simulink model "robot_2int_PI"  (R2024b)
settings: Solver=VariableStepAuto  StartTime=0.0  StopTime=10  RelTol=1e-3
values from neighbouring files (symbols this model uses):
  A_raid = diag([500, 500])    [solve_tp1.m]
  B_raid = diag([3000, 3000])    [solve_tp1.m]
  f_d = [10; 0]    [solve_tp1.m]
  K_raid = diag([2500, 2500])    [solve_tp1.m]
  Ke_raid = diag([10^4, 0])    [solve_tp1.m]
  ki = kp    (= 0.09)    [solve_tp1.m]
  kp = 9*10^-2    (= 0.09)    [solve_tp1.m]
libraries: slpidlib x1
settings Model: Creator=yago.milagres-passos  LastModifiedBy=yagom

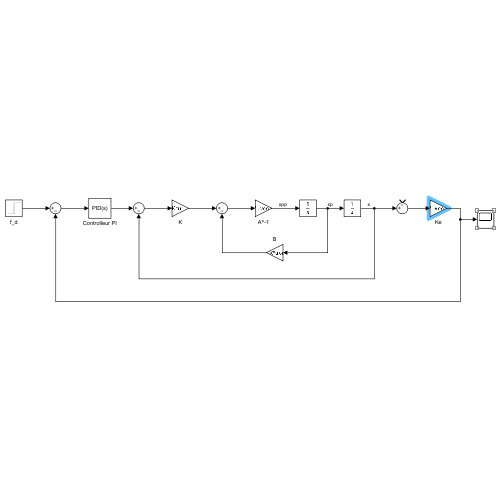
[thumbnail: Simulink's stored preview of the top-level diagram]
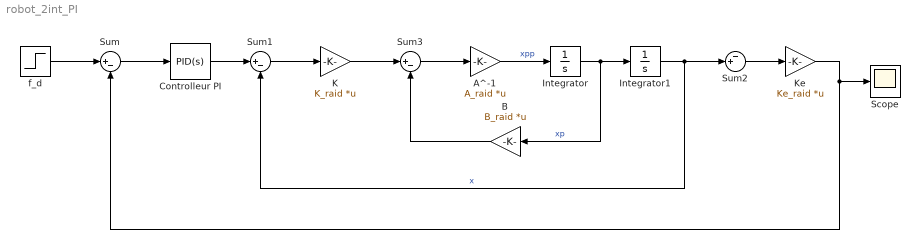
== system robot_2int_PI ==
  A^-1 : Gain  Gain=A_raid  Multiplication=Matrix(K*u) (u vector)
  B : Gain  Gain=B_raid  Multiplication=Matrix(K*u) (u vector)
  Controlleur PI : slpidlib/PID Controller  Controller=PID  Form=Parallel  TimeDomain=Continuous-time  UseExternalTs=off  SampleTime=-1  IntegratorMethod=Forward Euler  FilterMethod=Forward Euler  ControllerParametersSource=internal  P=kp  I=ki  UseKiTs=off  D=0  UseExternalDerivativeSource=off  N=100  UseFilter=on  TunerSelectOption=Transfer Function Based (PID Tuner App)  InitialConditionSource=internal  InitialConditionForIntegrator=0  InitialConditionForFilter=0  DifferentiatorICPrevScaledInput=0  ExternalReset=none  TrackingMode=off  Kt=1  LimitOutput=off  SatLimitsSource=internal  UpperSaturationLimit=inf  LowerSaturationLimit=-inf  LinearizeAsGain=on  AntiWindupMode=none  Kb=1  LimitIntegrator=off  UpperIntegratorSaturationLimit=inf  LowerIntegratorSaturationLimit=-inf  POutMin=[]  POutMax=[]  IOutMin=[]  IOutMax=[]  DOutMin=[]  DOutMax=[]  NOutMin=[]  NOutMax=[]  SumOutMin=[]  SumOutMax=[]  SaturationOutMin=[]  SaturationOutMax=[]  PParamMin=[]  PParamMax=[]  IParamMin=[]  IParamMax=[]  DParamMin=[]  DParamMax=[]  NParamMin=[]  NParamMax=[]  KbParamMin=[]  KbParamMax=[]  KtParamMin=[]  KtParamMax=[]  KbOutMin=[]  KbOutMax=[]  KtOutMin=[]  KtOutMax=[]  IntegratorOutMin=[]  IntegratorOutMax=[]  FilterOutMin=[]  FilterOutMax=[]  SumI1OutMin=[]  SumI1OutMax=[]  SumI2OutMin=[]  SumI2OutMax=[]  SumI3OutMin=[]  SumI3OutMax=[]  SumI4OutMin=[]  SumI4OutMax=[]  SumDOutMin=[]  SumDOutMax=[]  DifferentiatorOutMin=[]  DifferentiatorOutMax=[]  FilterDiffOutCoefMin=[]  FilterDiffOutCoefMax=[]  ReciprocalOutMin=[]  ReciprocalOutMax=[]  SumDenOutMin=[]  SumDenOutMax=[]  SumNumOutMin=[]  SumNumOutMax=[]  DivideOutMin=[]  DivideOutMax=[]  UdiffTsProdOutMin=[]  UdiffTsProdOutMax=[]  NTsProdOutMin=[]  NTsProdOutMax=[]  UintegralTsProdOutMin=[]  UintegralTsProdOutMax=[]  UngainTsProdOutMin=[]  UngainTsProdOutMax=[]  ClampingZeroOutDataTypeStr=Inherit: Inherit via back propagation  ClampingZeroOutMin=[]  ClampingZeroOutMax=[]  FilterDenConstantOutDataTypeStr=Inherit: Inherit via back propagation  FilterDenConstantOutMin=[]  FilterDenConstantOutMax=[]  PCopyOutDataTypeStr=Inherit: Inherit via back propagation  PCopyOutMin=[]  PCopyOutMax=[]  NCopyOutDataTypeStr=Inherit: Inherit via back propagation  NCopyOutMin=[]  NCopyOutMax=[]  IntegratorContinuousStateAttributes=''  IntegratorStateMustResolveToSignalObject=off  IntegratorRTWStateStorageClass=Auto  FilterContinuousStateAttributes=''  FilterStateMustResolveToSignalObject=off  FilterRTWStateStorageClass=Auto  ParallelPVariant=InternalParameters  IdealPVariant=Disabled  IVariant=InternalParameters  DVariant=InternalParameters  IntegratorVariant=Continuous  SatVariant=Disabled  AWVariant=Passthrough  PCopyVariant=Disabled  TRVariant=Disabled  FdbkBlocksVariant=Forward  IdealPFdbkVariant=Disabled  SatFdbkVariant=Disabled  DerivativeFilterVariant=ContFilter  NVariant=InternalParameters  NCopyVariant=Disabled  FilterICVariant=InternalICsFilter  IntegratorICVariant=InternalICs  ExternalResetVariant=Disabled  TRSumVariant=Passthrough  SumFdbkVariant=Disabled  SumVariant=Sum_PID  TsampFilterVariant=InternalTs  TsampNgainVariant=Passthrough  TsampIntegralVariant=Disabled_SignalSpec  ExternalSaturationOutDataTypeStr=Inherit: Same as second input  DerivativeSourceVariant=ErrorSignal  PreIntVariant=InternalPreInt
  Integrator : Integrator
  Integrator1 : Integrator
  K : Gain  Gain=K_raid  Multiplication=Matrix(K*u)
  Ke : Gain  Gain=Ke_raid  Multiplication=Matrix(K*u) (u vector)
  Scope : Scope
  Sum : Sum  Inputs=|+-
  Sum1 : Sum  Inputs=|+-
  Sum2 : Sum  Inputs=-+|
  Sum3 : Sum  Inputs=|+-
  f_d : Step  After=f_d  SampleTime=0
  wires:
  f_d/1 -> Sum/1
  Sum/1 -> Controlleur PI/1
  Sum1/1 -> K/1
  A^-1/1 -> Integrator/1  "xpp"
  Integrator/1 -> B/1, Integrator1/1  "xp"
  Integrator1/1 -> Sum1/2, Sum2/2  "x"
  Sum2/1 -> Ke/1
  K/1 -> Sum3/1
  Sum3/1 -> A^-1/1
  B/1 -> Sum3/2
  Ke/1 -> Sum/2, Scope/1
  Controlleur PI/1 -> Sum1/1
